simulink model "WindFarmDFIG"  (R2024a)
settings: Solver=FixedStepDiscrete  StartTime=0.0  StopTime=0.2  RelTol=1e-3
PreLoadFcn:
  | Ts=5e-6;
InitFcn:
  | xInitial = WindFarmDFIGInit;
  | Ts=5e-6;
undefined symbols (not defined in the file): D1, D11, Delta, DiscIntNeverNeededParam, find_system, level
libraries: powerlib_extras x38, spsThreePhaseVIMeasurementLib x6, simulink_extras x6, spsThreePhaseTransformerTwoWindingsLib x3, spsSeriesRLCBranchLib x2, spsUniversalBridgeLib x2, spsGroundLib x2, spsThreePhaseProgrammableVoltageSourceLib x1, spsThreePhaseMutualInductanceZ1Z0Lib x1, spsThreePhasePISectionLineLib x1, spsAsynchronousMachinepuUnitsLib x1, spsThreePhaseSeriesRLCBranchLib x1
(part 3 of 3)

== system WindFarmDFIG/DFIG Wind Turbine/Control/Measurement and Transformation/Discrete 3-phase PLL-Driven Positive-Sequence Active & Reactive Power/Discrete 3-phase PLL-Driven Positive-Sequence Fundamental Value/Discrete Variable Frequency Mean value1 ==
  note: Pierre Giroux, Gilbert Sybille, Richard Gagnon
      | Power System Simulation Laboratory
      | IREQ, Hydro-Quebc
  note: Variable frequency - Discrete Mean Value
  Freq : Inport  PortDimensions=1
  In : Inport  Port=2  PortDimensions=1
  Correction subsystem : Subsystem
  Discrete Variable Transport Delay : Subsystem  mask(Discrete variable transport delay){MaxDelay=MaxDelay, InitialValue=0, Ts=Ts}
      mask prompts: MaxDelay "Maximum delay (s):"; InitialValue "Initial input:"; Ts "Sample time:"
      mask help:
      | Apply a delay to the first input (In) signal.
      | The second input (D) specifies the delay time.
  Gain : Gain  Gain=Ts  SaturateOnIntegerOverflow=on  OutDataTypeStr=Inherit: Same as input  ParamDataTypeStr=Inherit: Same as input
  Integ4 : DiscreteIntegrator  IntegratorMethod=Integration: Trapezoidal  SampleTime=Ts  ICPrevOutput=DiscIntNeverNeededParam  ICPrevScaledInput=DiscIntNeverNeededParam
  Number of samples per cycle : Fcn  Expr=1/u[1]/Ts
  Product : Product  InputSameDT=on  SaturateOnIntegerOverflow=on  OutDataTypeStr=Inherit: Same as first input
  Rounding Function : Rounding  Operator=ceil
  Step : Step  Time=1/Finit  SampleTime=Ts
  Sum5 : Sum  InputSameDT=on  SaturateOnIntegerOverflow=on  OutDataTypeStr=Inherit: Same as first input
  Sum7 : Sum  Inputs=-+  InputSameDT=on  SaturateOnIntegerOverflow=on  OutDataTypeStr=Inherit: Same as first input
  Switch : Switch  Threshold=0.5  SaturateOnIntegerOverflow=off
  To avoid division by zero : Saturate  UpperLimit=1e6  LowerLimit=1e-6
  Unit Delay : UnitDelay  InitialCondition=Vinit  SampleTime=Ts  HasFrameUpgradeWarning=on
  Mean : Outport  VectorParamsAs1DForOutWhenUnconnected=off
  wires:
  In/1 -> Integ4/1, Correction subsystem/3(In)  "In"
  Product/1 -> Sum5/1  "Mean value"
  Discrete Variable Transport Delay/1(Out) -> Sum7/1
  Sum7/1 -> Product/1
  Integ4/1 -> Discrete Variable Transport Delay/1(In), Sum7/2
  Freq/1 -> Product/2, To avoid division by zero/1  "Freq"
  Gain/1 -> Discrete Variable Transport Delay/2(D)  "Delay"
  Rounding Function/1 -> Gain/1, Correction subsystem/2(F)
  Number of samples per cycle/1 -> Rounding Function/1, Correction subsystem/1(N)
  Sum5/1 -> Switch/1
  Unit Delay/1 -> Switch/3
  Switch/1 -> Mean/1, Unit Delay/1
  To avoid division by zero/1 -> Number of samples per cycle/1  "Freq"
  Correction subsystem/1(Out) -> Sum5/2
  Step/1 -> Switch/2

== system WindFarmDFIG/DFIG Wind Turbine/Control/Measurement and Transformation/Discrete 3-phase PLL-Driven Positive-Sequence Active & Reactive Power/Discrete 3-phase PLL-Driven Positive-Sequence Fundamental Value/Discrete Variable Frequency Mean value2 ==
  note: Variable frequency - Discrete Mean Value
  note: Pierre Giroux, Gilbert Sybille, Richard Gagnon
      | Power System Simulation Laboratory
      | IREQ, Hydro-Quebc
  Freq : Inport  PortDimensions=1
  In : Inport  Port=2  PortDimensions=1
  Correction subsystem : Subsystem
  Discrete Variable Transport Delay : Subsystem  mask(Discrete variable transport delay){MaxDelay=MaxDelay, InitialValue=0, Ts=Ts}
      mask prompts: MaxDelay "Maximum delay (s):"; InitialValue "Initial input:"; Ts "Sample time:"
      mask help:
      | Apply a delay to the first input (In) signal.
      | The second input (D) specifies the delay time.
  Gain : Gain  Gain=Ts  SaturateOnIntegerOverflow=on  OutDataTypeStr=Inherit: Same as input  ParamDataTypeStr=Inherit: Same as input
  Integ4 : DiscreteIntegrator  IntegratorMethod=Integration: Trapezoidal  SampleTime=Ts  ICPrevOutput=DiscIntNeverNeededParam  ICPrevScaledInput=DiscIntNeverNeededParam
  Number of samples per cycle : Fcn  Expr=1/u[1]/Ts
  Product : Product  InputSameDT=on  SaturateOnIntegerOverflow=on  OutDataTypeStr=Inherit: Same as first input
  Rounding Function : Rounding  Operator=ceil
  Step : Step  Time=1/Finit  SampleTime=Ts
  Sum5 : Sum  InputSameDT=on  SaturateOnIntegerOverflow=on  OutDataTypeStr=Inherit: Same as first input
  Sum7 : Sum  Inputs=-+  InputSameDT=on  SaturateOnIntegerOverflow=on  OutDataTypeStr=Inherit: Same as first input
  Switch : Switch  Threshold=0.5  SaturateOnIntegerOverflow=off
  To avoid division by zero : Saturate  UpperLimit=1e6  LowerLimit=1e-6
  Unit Delay : UnitDelay  InitialCondition=Vinit  SampleTime=Ts  HasFrameUpgradeWarning=on
  Mean : Outport  VectorParamsAs1DForOutWhenUnconnected=off
  wires:
  Step/1 -> Switch/2
  Correction subsystem/1(Out) -> Sum5/2
  To avoid division by zero/1 -> Number of samples per cycle/1  "Freq"
  Switch/1 -> Unit Delay/1, Mean/1
  Unit Delay/1 -> Switch/3
  Sum5/1 -> Switch/1
  Number of samples per cycle/1 -> Correction subsystem/1(N), Rounding Function/1
  Rounding Function/1 -> Correction subsystem/2(F), Gain/1
  Gain/1 -> Discrete Variable Transport Delay/2(D)  "Delay"
  Freq/1 -> To avoid division by zero/1, Product/2  "Freq"
  Integ4/1 -> Sum7/2, Discrete Variable Transport Delay/1(In)
  Sum7/1 -> Product/1
  Discrete Variable Transport Delay/1(Out) -> Sum7/1
  Product/1 -> Sum5/1  "Mean value"
  In/1 -> Correction subsystem/3(In), Integ4/1  "In"

== system WindFarmDFIG/DFIG Wind Turbine/Control/Measurement and Transformation/Discrete 3-phase PLL-Driven Positive-Sequence Active & Reactive Power/Discrete 3-phase PLL-Driven Positive-Sequence Fundamental Value2/Discrete Variable Frequency Mean value1 ==
  note: Variable frequency - Discrete Mean Value
  note: Pierre Giroux, Gilbert Sybille, Richard Gagnon
      | Power System Simulation Laboratory
      | IREQ, Hydro-Quebc
  Freq : Inport  PortDimensions=1
  In : Inport  Port=2  PortDimensions=1
  Correction subsystem : Subsystem
  Discrete Variable Transport Delay : Subsystem  mask(Discrete variable transport delay){MaxDelay=MaxDelay, InitialValue=0, Ts=Ts}
      mask prompts: MaxDelay "Maximum delay (s):"; InitialValue "Initial input:"; Ts "Sample time:"
      mask help:
      | Apply a delay to the first input (In) signal.
      | The second input (D) specifies the delay time.
  Gain : Gain  Gain=Ts  SaturateOnIntegerOverflow=on  OutDataTypeStr=Inherit: Same as input  ParamDataTypeStr=Inherit: Same as input
  Integ4 : DiscreteIntegrator  IntegratorMethod=Integration: Trapezoidal  SampleTime=Ts  ICPrevOutput=DiscIntNeverNeededParam  ICPrevScaledInput=DiscIntNeverNeededParam
  Number of samples per cycle : Fcn  Expr=1/u[1]/Ts
  Product : Product  InputSameDT=on  SaturateOnIntegerOverflow=on  OutDataTypeStr=Inherit: Same as first input
  Rounding Function : Rounding  Operator=ceil
  Step : Step  Time=1/Finit  SampleTime=Ts
  Sum5 : Sum  InputSameDT=on  SaturateOnIntegerOverflow=on  OutDataTypeStr=Inherit: Same as first input
  Sum7 : Sum  Inputs=-+  InputSameDT=on  SaturateOnIntegerOverflow=on  OutDataTypeStr=Inherit: Same as first input
  Switch : Switch  Threshold=0.5  SaturateOnIntegerOverflow=off
  To avoid division by zero : Saturate  UpperLimit=1e6  LowerLimit=1e-6
  Unit Delay : UnitDelay  InitialCondition=Vinit  SampleTime=Ts  HasFrameUpgradeWarning=on
  Mean : Outport  VectorParamsAs1DForOutWhenUnconnected=off
  wires:
  Step/1 -> Switch/2
  Correction subsystem/1(Out) -> Sum5/2
  To avoid division by zero/1 -> Number of samples per cycle/1  "Freq"
  Switch/1 -> Unit Delay/1, Mean/1
  Unit Delay/1 -> Switch/3
  Sum5/1 -> Switch/1
  Number of samples per cycle/1 -> Correction subsystem/1(N), Rounding Function/1
  Rounding Function/1 -> Correction subsystem/2(F), Gain/1
  Gain/1 -> Discrete Variable Transport Delay/2(D)  "Delay"
  Freq/1 -> To avoid division by zero/1, Product/2  "Freq"
  Integ4/1 -> Sum7/2, Discrete Variable Transport Delay/1(In)
  Sum7/1 -> Product/1
  Discrete Variable Transport Delay/1(Out) -> Sum7/1
  Product/1 -> Sum5/1  "Mean value"
  In/1 -> Correction subsystem/3(In), Integ4/1  "In"

== system WindFarmDFIG/DFIG Wind Turbine/Control/Measurement and Transformation/Discrete 3-phase PLL-Driven Positive-Sequence Active & Reactive Power/Discrete 3-phase PLL-Driven Positive-Sequence Fundamental Value2/Discrete Variable Frequency Mean value2 ==
  note: Pierre Giroux, Gilbert Sybille, Richard Gagnon
      | Power System Simulation Laboratory
      | IREQ, Hydro-Quebc
  note: Variable frequency - Discrete Mean Value
  Freq : Inport  PortDimensions=1
  In : Inport  Port=2  PortDimensions=1
  Correction subsystem : Subsystem
  Discrete Variable Transport Delay : Subsystem  mask(Discrete variable transport delay){MaxDelay=MaxDelay, InitialValue=0, Ts=Ts}
      mask prompts: MaxDelay "Maximum delay (s):"; InitialValue "Initial input:"; Ts "Sample time:"
      mask help:
      | Apply a delay to the first input (In) signal.
      | The second input (D) specifies the delay time.
  Gain : Gain  Gain=Ts  SaturateOnIntegerOverflow=on  OutDataTypeStr=Inherit: Same as input  ParamDataTypeStr=Inherit: Same as input
  Integ4 : DiscreteIntegrator  IntegratorMethod=Integration: Trapezoidal  SampleTime=Ts  ICPrevOutput=DiscIntNeverNeededParam  ICPrevScaledInput=DiscIntNeverNeededParam
  Number of samples per cycle : Fcn  Expr=1/u[1]/Ts
  Product : Product  InputSameDT=on  SaturateOnIntegerOverflow=on  OutDataTypeStr=Inherit: Same as first input
  Rounding Function : Rounding  Operator=ceil
  Step : Step  Time=1/Finit  SampleTime=Ts
  Sum5 : Sum  InputSameDT=on  SaturateOnIntegerOverflow=on  OutDataTypeStr=Inherit: Same as first input
  Sum7 : Sum  Inputs=-+  InputSameDT=on  SaturateOnIntegerOverflow=on  OutDataTypeStr=Inherit: Same as first input
  Switch : Switch  Threshold=0.5  SaturateOnIntegerOverflow=off
  To avoid division by zero : Saturate  UpperLimit=1e6  LowerLimit=1e-6
  Unit Delay : UnitDelay  InitialCondition=Vinit  SampleTime=Ts  HasFrameUpgradeWarning=on
  Mean : Outport  VectorParamsAs1DForOutWhenUnconnected=off
  wires:
  In/1 -> Integ4/1, Correction subsystem/3(In)  "In"
  Product/1 -> Sum5/1  "Mean value"
  Discrete Variable Transport Delay/1(Out) -> Sum7/1
  Sum7/1 -> Product/1
  Integ4/1 -> Discrete Variable Transport Delay/1(In), Sum7/2
  Freq/1 -> Product/2, To avoid division by zero/1  "Freq"
  Gain/1 -> Discrete Variable Transport Delay/2(D)  "Delay"
  Rounding Function/1 -> Gain/1, Correction subsystem/2(F)
  Number of samples per cycle/1 -> Rounding Function/1, Correction subsystem/1(N)
  Sum5/1 -> Switch/1
  Unit Delay/1 -> Switch/3
  Switch/1 -> Mean/1, Unit Delay/1
  To avoid division by zero/1 -> Number of samples per cycle/1  "Freq"
  Correction subsystem/1(Out) -> Sum5/2
  Step/1 -> Switch/2

== system WindFarmDFIG/DFIG Wind Turbine/Control/Measurement and Transformation/Discrete 3-phase PLL-Driven Positive-Sequence Active & Reactive Power/Discrete 3-phase PLL-Driven Positive-Sequence Fundamental Value/Discrete Variable Frequency Mean value1/Correction subsystem ==
  N : Inport
  F : Inport  Port=2
  In : Inport  Port=3
  Gain1 : Gain  Gain=0.5  SaturateOnIntegerOverflow=on  OutDataTypeStr=Inherit: Same as input  ParamDataTypeStr=Inherit: Same as input
  Product2 : Product  Inputs=*/  InputSameDT=on  SaturateOnIntegerOverflow=on  OutDataTypeStr=Inherit: Same as first input
  Product4 : Product  Inputs=**  InputSameDT=on  SaturateOnIntegerOverflow=on  OutDataTypeStr=Inherit: Same as first input
  Product5 : Product  Inputs=**  InputSameDT=on  SaturateOnIntegerOverflow=on  OutDataTypeStr=Inherit: Same as first input
  Sum1 : Sum  Inputs=+-  InputSameDT=on  SaturateOnIntegerOverflow=on  OutDataTypeStr=Inherit: Same as first input
  Sum4 : Sum  InputSameDT=on  SaturateOnIntegerOverflow=on  OutDataTypeStr=Inherit: Same as first input
  Sum5 : Sum  Inputs=+-  InputSameDT=on  SaturateOnIntegerOverflow=on  OutDataTypeStr=Inherit: Same as first input
  Unit Delay : UnitDelay  SampleTime=Ts  HasFrameUpgradeWarning=on
  Out : Outport  VectorParamsAs1DForOutWhenUnconnected=off
  wires:
  Unit Delay/1 -> Sum1/2
  N/1 -> Sum5/1, Product2/2
  F/1 -> Sum5/2
  Sum5/1 -> Product2/1, Product5/1
  Product2/1 -> Product4/1
  In/1 -> Sum1/1, Unit Delay/1, Sum4/2
  Sum1/1 -> Product5/2
  Product5/1 -> Gain1/1
  Gain1/1 -> Sum4/1
  Sum4/1 -> Product4/2
  Product4/1 -> Out/1

== system WindFarmDFIG/DFIG Wind Turbine/Control/Measurement and Transformation/Discrete 3-phase PLL-Driven Positive-Sequence Active & Reactive Power/Discrete 3-phase PLL-Driven Positive-Sequence Fundamental Value/Discrete Variable Frequency Mean value1/Discrete Variable Transport Delay ==
  In : Inport
  D : Inport  Port=2
  "S-Function " : S-Function  FunctionName=discreteVariableTransportDelay  Parameters=MaxDelay,Ts,InitialValue  SFunctionDeploymentMode=off  EnableBusSupport=off
  Out : Outport  VectorParamsAs1DForOutWhenUnconnected=off
  wires:
  "S-Function "/1 -> Out/1
  In/1 -> "S-Function "/1
  D/1 -> "S-Function "/2

== system WindFarmDFIG/DFIG Wind Turbine/Control/Measurement and Transformation/Discrete 3-phase PLL-Driven Positive-Sequence Active & Reactive Power/Discrete 3-phase PLL-Driven Positive-Sequence Fundamental Value/Discrete Variable Frequency Mean value2/Correction subsystem ==
  N : Inport
  F : Inport  Port=2
  In : Inport  Port=3
  Gain1 : Gain  Gain=0.5  SaturateOnIntegerOverflow=on  OutDataTypeStr=Inherit: Same as input  ParamDataTypeStr=Inherit: Same as input
  Product2 : Product  Inputs=*/  InputSameDT=on  SaturateOnIntegerOverflow=on  OutDataTypeStr=Inherit: Same as first input
  Product4 : Product  Inputs=**  InputSameDT=on  SaturateOnIntegerOverflow=on  OutDataTypeStr=Inherit: Same as first input
  Product5 : Product  Inputs=**  InputSameDT=on  SaturateOnIntegerOverflow=on  OutDataTypeStr=Inherit: Same as first input
  Sum1 : Sum  Inputs=+-  InputSameDT=on  SaturateOnIntegerOverflow=on  OutDataTypeStr=Inherit: Same as first input
  Sum4 : Sum  InputSameDT=on  SaturateOnIntegerOverflow=on  OutDataTypeStr=Inherit: Same as first input
  Sum5 : Sum  Inputs=+-  InputSameDT=on  SaturateOnIntegerOverflow=on  OutDataTypeStr=Inherit: Same as first input
  Unit Delay : UnitDelay  SampleTime=Ts  HasFrameUpgradeWarning=on
  Out : Outport  VectorParamsAs1DForOutWhenUnconnected=off
  wires:
  Product4/1 -> Out/1
  Sum4/1 -> Product4/2
  Gain1/1 -> Sum4/1
  Product5/1 -> Gain1/1
  Sum1/1 -> Product5/2
  In/1 -> Sum4/2, Unit Delay/1, Sum1/1
  Product2/1 -> Product4/1
  Sum5/1 -> Product5/1, Product2/1
  F/1 -> Sum5/2
  N/1 -> Product2/2, Sum5/1
  Unit Delay/1 -> Sum1/2

== system WindFarmDFIG/DFIG Wind Turbine/Control/Measurement and Transformation/Discrete 3-phase PLL-Driven Positive-Sequence Active & Reactive Power/Discrete 3-phase PLL-Driven Positive-Sequence Fundamental Value/Discrete Variable Frequency Mean value2/Discrete Variable Transport Delay ==
  In : Inport
  D : Inport  Port=2
  "S-Function " : S-Function  FunctionName=discreteVariableTransportDelay  Parameters=MaxDelay,Ts,InitialValue  SFunctionDeploymentMode=off  EnableBusSupport=off
  Out : Outport  VectorParamsAs1DForOutWhenUnconnected=off
  wires:
  D/1 -> "S-Function "/2
  In/1 -> "S-Function "/1
  "S-Function "/1 -> Out/1

== system WindFarmDFIG/DFIG Wind Turbine/Control/Measurement and Transformation/Discrete 3-phase PLL-Driven Positive-Sequence Active & Reactive Power/Discrete 3-phase PLL-Driven Positive-Sequence Fundamental Value2/Discrete Variable Frequency Mean value1/Correction subsystem ==
  N : Inport
  F : Inport  Port=2
  In : Inport  Port=3
  Gain1 : Gain  Gain=0.5  SaturateOnIntegerOverflow=on  OutDataTypeStr=Inherit: Same as input  ParamDataTypeStr=Inherit: Same as input
  Product2 : Product  Inputs=*/  InputSameDT=on  SaturateOnIntegerOverflow=on  OutDataTypeStr=Inherit: Same as first input
  Product4 : Product  Inputs=**  InputSameDT=on  SaturateOnIntegerOverflow=on  OutDataTypeStr=Inherit: Same as first input
  Product5 : Product  Inputs=**  InputSameDT=on  SaturateOnIntegerOverflow=on  OutDataTypeStr=Inherit: Same as first input
  Sum1 : Sum  Inputs=+-  InputSameDT=on  SaturateOnIntegerOverflow=on  OutDataTypeStr=Inherit: Same as first input
  Sum4 : Sum  InputSameDT=on  SaturateOnIntegerOverflow=on  OutDataTypeStr=Inherit: Same as first input
  Sum5 : Sum  Inputs=+-  InputSameDT=on  SaturateOnIntegerOverflow=on  OutDataTypeStr=Inherit: Same as first input
  Unit Delay : UnitDelay  SampleTime=Ts  HasFrameUpgradeWarning=on
  Out : Outport  VectorParamsAs1DForOutWhenUnconnected=off
  wires:
  Product4/1 -> Out/1
  Sum4/1 -> Product4/2
  Gain1/1 -> Sum4/1
  Product5/1 -> Gain1/1
  Sum1/1 -> Product5/2
  In/1 -> Sum4/2, Unit Delay/1, Sum1/1
  Product2/1 -> Product4/1
  Sum5/1 -> Product5/1, Product2/1
  F/1 -> Sum5/2
  N/1 -> Product2/2, Sum5/1
  Unit Delay/1 -> Sum1/2

== system WindFarmDFIG/DFIG Wind Turbine/Control/Measurement and Transformation/Discrete 3-phase PLL-Driven Positive-Sequence Active & Reactive Power/Discrete 3-phase PLL-Driven Positive-Sequence Fundamental Value2/Discrete Variable Frequency Mean value1/Discrete Variable Transport Delay ==
  In : Inport
  D : Inport  Port=2
  "S-Function " : S-Function  FunctionName=discreteVariableTransportDelay  Parameters=MaxDelay,Ts,InitialValue  SFunctionDeploymentMode=off  EnableBusSupport=off
  Out : Outport  VectorParamsAs1DForOutWhenUnconnected=off
  wires:
  D/1 -> "S-Function "/2
  In/1 -> "S-Function "/1
  "S-Function "/1 -> Out/1

== system WindFarmDFIG/DFIG Wind Turbine/Control/Measurement and Transformation/Discrete 3-phase PLL-Driven Positive-Sequence Active & Reactive Power/Discrete 3-phase PLL-Driven Positive-Sequence Fundamental Value2/Discrete Variable Frequency Mean value2/Correction subsystem ==
  N : Inport
  F : Inport  Port=2
  In : Inport  Port=3
  Gain1 : Gain  Gain=0.5  SaturateOnIntegerOverflow=on  OutDataTypeStr=Inherit: Same as input  ParamDataTypeStr=Inherit: Same as input
  Product2 : Product  Inputs=*/  InputSameDT=on  SaturateOnIntegerOverflow=on  OutDataTypeStr=Inherit: Same as first input
  Product4 : Product  Inputs=**  InputSameDT=on  SaturateOnIntegerOverflow=on  OutDataTypeStr=Inherit: Same as first input
  Product5 : Product  Inputs=**  InputSameDT=on  SaturateOnIntegerOverflow=on  OutDataTypeStr=Inherit: Same as first input
  Sum1 : Sum  Inputs=+-  InputSameDT=on  SaturateOnIntegerOverflow=on  OutDataTypeStr=Inherit: Same as first input
  Sum4 : Sum  InputSameDT=on  SaturateOnIntegerOverflow=on  OutDataTypeStr=Inherit: Same as first input
  Sum5 : Sum  Inputs=+-  InputSameDT=on  SaturateOnIntegerOverflow=on  OutDataTypeStr=Inherit: Same as first input
  Unit Delay : UnitDelay  SampleTime=Ts  HasFrameUpgradeWarning=on
  Out : Outport  VectorParamsAs1DForOutWhenUnconnected=off
  wires:
  Unit Delay/1 -> Sum1/2
  N/1 -> Sum5/1, Product2/2
  F/1 -> Sum5/2
  Sum5/1 -> Product2/1, Product5/1
  Product2/1 -> Product4/1
  In/1 -> Sum1/1, Unit Delay/1, Sum4/2
  Sum1/1 -> Product5/2
  Product5/1 -> Gain1/1
  Gain1/1 -> Sum4/1
  Sum4/1 -> Product4/2
  Product4/1 -> Out/1

== system WindFarmDFIG/DFIG Wind Turbine/Control/Measurement and Transformation/Discrete 3-phase PLL-Driven Positive-Sequence Active & Reactive Power/Discrete 3-phase PLL-Driven Positive-Sequence Fundamental Value2/Discrete Variable Frequency Mean value2/Discrete Variable Transport Delay ==
  In : Inport
  D : Inport  Port=2
  "S-Function " : S-Function  FunctionName=discreteVariableTransportDelay  Parameters=MaxDelay,Ts,InitialValue  SFunctionDeploymentMode=off  EnableBusSupport=off
  Out : Outport  VectorParamsAs1DForOutWhenUnconnected=off
  wires:
  "S-Function "/1 -> Out/1
  In/1 -> "S-Function "/1
  D/1 -> "S-Function "/2
